simulink model "structure_plant"  (R2026b)
settings: Solver=VariableStepAuto
undefined symbols (not defined in the file or in its folder): P, Ts
settings Model: Creator=aomar  LastModifiedBy=aomar

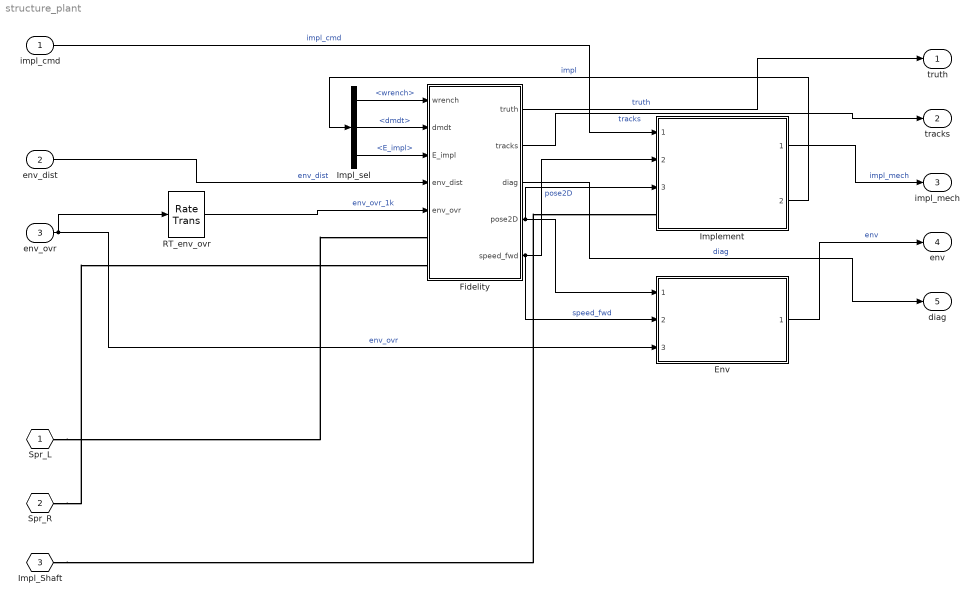
== system structure_plant ==
  impl_cmd : Inport  OutDataTypeStr=Bus: Bus_ImplementCmd  SampleTime=Ts.ctrl
  env_dist : Inport  Port=2  OutDataTypeStr=Bus: Bus_EnvDisturbance  SampleTime=Ts.base
  env_ovr : Inport  Port=3  OutDataTypeStr=Bus: Bus_EnvOverride  SampleTime=Ts.env
  Env : Subsystem  ReferencedSubsystem=structure_env
  Fidelity : Subsystem  Variant=on
  Impl_sel : BusSelector  OutputSignals=wrench,dmdt,E_impl
  Implement : Subsystem  ReferencedSubsystem=structure_implement
  RT_env_ovr : RateTransition  InitialCondition=P.ic.Bus_EnvOverride  OutPortSampleTime=Ts.base
  Spr_L : PMIOPort  Side=Left  ConnectionType=Connection: foundation.mechanical.rotational.rotational
  Spr_R : PMIOPort  Port=2  Side=Left  ConnectionType=Connection: foundation.mechanical.rotational.rotational
  Impl_Shaft : PMIOPort  Port=3  Side=Left  ConnectionType=Connection: foundation.mechanical.rotational.rotational
  truth : Outport  OutDataTypeStr=Bus: Bus_TruthState
  tracks : Outport  Port=2  OutDataTypeStr=Bus: Bus_TrackState
  impl_mech : Outport  Port=3  OutDataTypeStr=Bus: Bus_ImplMechState  SampleTime=Ts.ctrl
  env : Outport  Port=4  OutDataTypeStr=Bus: Bus_EnvState  SampleTime=Ts.env
  diag : Outport  Port=5  OutDataTypeStr=Bus: Bus_StructureDiag
  wires:
  impl_cmd/1 -> Implement/1  "impl_cmd"
  env_dist/1 -> Fidelity/4(env_dist)  "env_dist"
  env_ovr/1 -> Env/3, RT_env_ovr/1  "env_ovr"
  RT_env_ovr/1 -> Fidelity/5(env_ovr)  "env_ovr_1k"
  Impl_sel/1 -> Fidelity/1(wrench)  "<wrench>"
  Impl_sel/2 -> Fidelity/2(dmdt)  "<dmdt>"
  Impl_sel/3 -> Fidelity/3(E_impl)  "<E_impl>"
  Fidelity/1(truth) -> truth/1  "truth"
  Fidelity/2(tracks) -> tracks/1  "tracks"
  Fidelity/3(diag) -> diag/1  "diag"
  Fidelity/4(pose2D) -> Env/1, Implement/3  "pose2D"
  Fidelity/5(speed_fwd) -> Implement/2, Env/2  "speed_fwd"
  Implement/1 -> impl_mech/1  "impl_mech"
  Implement/2 -> Impl_sel/1  "impl"
  Env/1 -> env/1  "env"
  connections:
  Spr_L/RConn1 -- Fidelity/LConn1
  Spr_R/RConn1 -- Fidelity/LConn2
  Impl_Shaft/RConn1 -- Implement/LConn1

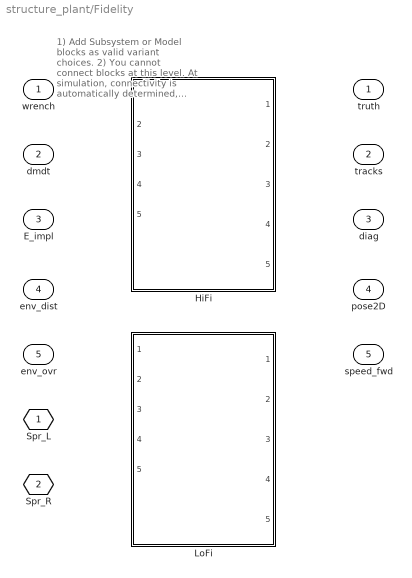
== system structure_plant/Fidelity ==
  note: 1) Add Subsystem or Model blocks as valid variant choices.
      | 2) You cannot connect blocks at this level. At simulation, connectivity is automatically
      | determined, based on the active variant and port name matching.
  wrench : Inport
  dmdt : Inport  Port=2
  E_impl : Inport  Port=3
  env_dist : Inport  Port=4  OutDataTypeStr=Bus: Bus_EnvDisturbance
  env_ovr : Inport  Port=5  OutDataTypeStr=Bus: Bus_EnvOverride
  HiFi : Subsystem  VariantControl=VC_STRUCT_FID == 1  ReferencedSubsystem=structure_hifi
  LoFi : Subsystem  VariantControl=VC_STRUCT_FID == 2  ReferencedSubsystem=structure_lofi
  Spr_L : PMIOPort  Side=Left  ConnectionType=Connection: foundation.mechanical.rotational.rotational
  Spr_R : PMIOPort  Port=2  Side=Left  ConnectionType=Connection: foundation.mechanical.rotational.rotational
  truth : Outport  OutDataTypeStr=Bus: Bus_TruthState
  tracks : Outport  Port=2  OutDataTypeStr=Bus: Bus_TrackState
  diag : Outport  Port=3  OutDataTypeStr=Bus: Bus_StructureDiag
  pose2D : Outport  Port=4
  speed_fwd : Outport  Port=5
